simulink model "digital_modlation"  (R2025a)
settings: Solver=VariableStepAuto  StartTime=0.0  StopTime=1  RelTol=1e-3
libraries: dspfdesign x2, commdigbbndpm3 x2, commchan3 x1, commrandsrc3 x1
settings Model: Creator=user  LastModifiedBy=LaL
settings RTWCC: GPUComputeCapability=3.5

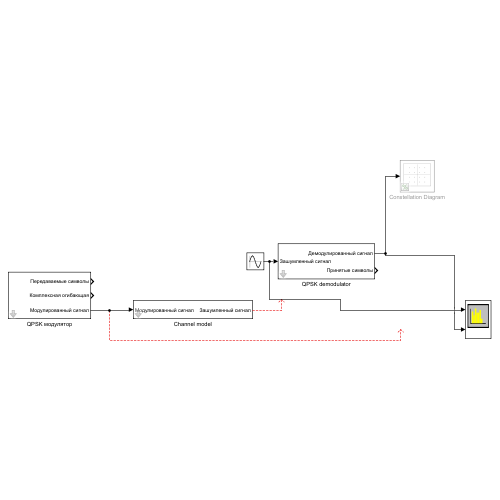
[thumbnail: Simulink's stored preview of the top-level diagram]
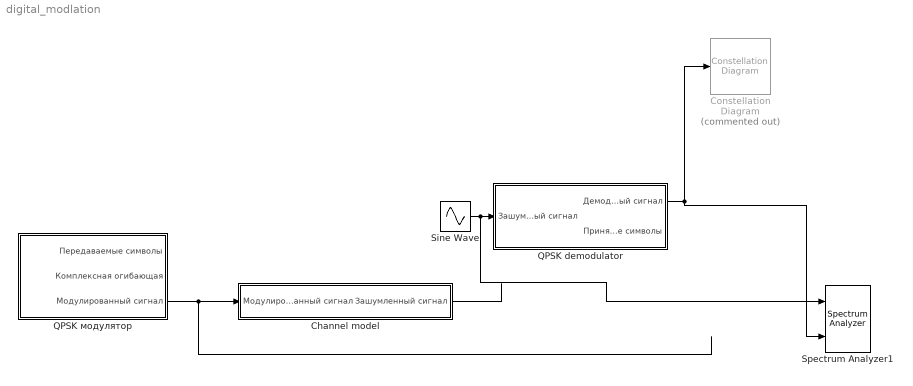
== system digital_modlation ==
  Channel model : Subsystem  mask{SNR=20}
      mask prompts: SNR "SNR (dB)"
  Constellation Diagram : ConstellationDiagram  Commented=on  WindowPosition=[452.000000,103.000000,600.000000,600.000000,]  ScopeFrameLocation=window  SymbolsToDisplaySource=Property  SymbolsToDisplay=300  XLimits=[-1.46,1.46]  YLimits=[-1.38,1.38]  AxesLimits=[-1.38,1.38]  DefaultConfigurationName=comm.scopes.ConstellationDiagramBlockCfg
  QPSK demodulator : Subsystem  mask{symspeed=1000, f=10000, f_d=100000}
      mask prompts: symspeed "Символьная скорость"; f "Частота несущей"; f_d "Частота дискретизации"
  QPSK модулятор : Subsystem  mask{symspeed=1000, f=10000, f_d=100000}
      mask prompts: symspeed "Символьная скорость"; f "Частота несущей"; f_d "Частота дискретизации"
  Sine Wave : Sin  Frequency=10000
  Spectrum Analyzer1 : SpectrumAnalyzer  NumInputPorts=2  WindowPosition=[495.000000,168.000000,800.000000,500.000000,]  Visible=on  ScopeFrameLocation=window  Span=99999.99999999999  StartFrequency=-49999.99999999999  StopFrequency=49999.99999999999  YLimits=[-236.26963761,59.54612507]  SelectedToolstripTab=spectrumAnalyzerToolstrip.measurementsTab
  wires:
  QPSK модулятор/3(Модулированный сигнал) -> Channel model/1(Модулированный сигнал)
  Channel model/1(Зашумленный сигнал) -> ?
  QPSK demodulator/1(Демодулированный сигнал) -> Constellation Diagram/1, Spectrum Analyzer1/2
  Sine Wave/1 -> Spectrum Analyzer1/1, QPSK demodulator/1(Зашумленный сигнал)

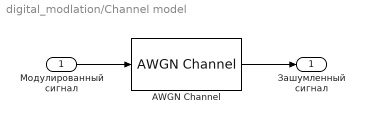
== system digital_modlation/Channel model ==
  Модулированный сигнал : Inport
  AWGN Channel : commchan3/AWGN Channel  LegacyMode=off  NoiseMethod="Signal to noise ratio  (SNR)"  noiseMode="Signal to noise ratio  (SNR)"  EbNo=10  EsNo=10  SNR=SNR  BitsPerSymbol=1  SignalPower=1  SamplesPerSymbol=1  SymbolPeriod=1  VarianceSource=Parameter  Variance=1  RandomStream=Global stream  Seed=67  SimulateUsing=Code generation
  Зашумленный сигнал : Outport
  wires:
  Модулированный сигнал/1 -> AWGN Channel/1
  AWGN Channel/1 -> Зашумленный сигнал/1

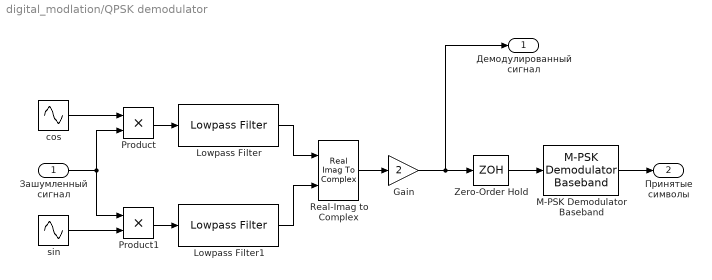
== system digital_modlation/QPSK demodulator ==
  Зашумленный сигнал : Inport
  Gain : Gain  Gain=2
  Lowpass Filter : dspfdesign/Lowpass Filter  FilterType=FIR  DesignForMinimumOrder=on  FilterOrder=50  PassbandFrequency=f  StopbandFrequency=1.2*f  PassbandRipple=0.1  StopbandAttenuation=80  SampleRateMode=Specify on dialog  SampleRate=f_d  SimulateUsing=Interpreted execution  roundingMode=Floor  coeffsDataTypeStr=fixdt(1,16)
  Lowpass Filter1 : dspfdesign/Lowpass Filter  FilterType=FIR  DesignForMinimumOrder=on  FilterOrder=50  PassbandFrequency=f  StopbandFrequency=1.2*f  PassbandRipple=0.1  StopbandAttenuation=80  SampleRateMode=Specify on dialog  SampleRate=f_d  SimulateUsing=Interpreted execution  roundingMode=Floor  coeffsDataTypeStr=fixdt(1,16)
  M-PSK Demodulator Baseband : commdigbbndpm3/M-PSK Demodulator Baseband  M=4  OutType=Integer  DecType=Hard decision  VarSource=Dialog  Variance=1  Dec=Gray  Mapping=[0:7]  Ph=pi/4  outDtype1=Inherit via internal rule  outDtype2=Inherit via internal rule  derotateFactorWordLen=16  derotateFactorDataTypeStr=Inherit: Same word length as input  derotateFactorLastDataTypeStr=Inherit: Same word length as input
      settings: LibrarySourceBlock=|
      | commhdldigbbndpm/M-PSK
      | Demodulator
      | Baseband
  Product : Product
  Product1 : Product
  Real-Imag to Complex : RealImagToComplex
  Zero-Order Hold : ZeroOrderHold  SampleTime=1/symspeed
  cos : Sin  Frequency=2*pi*f  Phase=pi/2  SampleTime=1/f_d
  sin : Sin  Frequency=2*pi*f  SampleTime=1/f_d
  Демодулированный сигнал : Outport
  Принятые символы : Outport  Port=2
  wires:
  Зашумленный сигнал/1 -> Product/2, Product1/1
  cos/1 -> Product/1
  sin/1 -> Product1/2
  Product/1 -> Lowpass Filter/1
  Product1/1 -> Lowpass Filter1/1
  Lowpass Filter/1 -> Real-Imag to Complex/1
  Lowpass Filter1/1 -> Real-Imag to Complex/2
  Real-Imag to Complex/1 -> Gain/1
  Gain/1 -> Zero-Order Hold/1, Демодулированный сигнал/1
  Zero-Order Hold/1 -> M-PSK Demodulator Baseband/1
  M-PSK Demodulator Baseband/1 -> Принятые символы/1

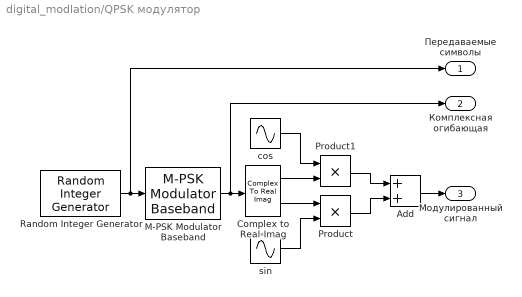
== system digital_modlation/QPSK модулятор ==
  Add : Sum
  Complex to Real-Imag : ComplexToRealImag
  M-PSK Modulator Baseband : commdigbbndpm3/M-PSK Modulator Baseband  M=4  InType=Integer  Enc=Gray  Mapping=[0:7]  Ph=pi/4  outDtype=double  outWordLen=16  outUDDataType=sfix(16)  outFracLenMode=Best precision  outFracLen=15  outDataTypeStr=double  outLastDataTypeStr=double
      settings: LibrarySourceBlock=|
      | commhdldigbbndpm/M-PSK
      | Modulator
      | Baseband
  Product : Product
  Product1 : Product
  Random Integer Generator : commrandsrc3/Random Integer Generator  SetSize=4  SeedSource=Auto  Seed=0  SampleTime=1/symspeed  SamplesPerFrame=1  OutputDataType=uint8  SimulateUsing=Interpreted execution
  cos : Sin  Frequency=2*pi*f  Phase=pi/2  SampleTime=1/f_d
  sin : Sin  Frequency=2*pi*f  SampleTime=1/f_d
  Передаваемые символы : Outport
  Комплексная огибающая : Outport  Port=2
  Модулированный сигнал : Outport  Port=3
  wires:
  Random Integer Generator/1 -> Передаваемые символы/1, M-PSK Modulator Baseband/1
  M-PSK Modulator Baseband/1 -> Комплексная огибающая/1, Complex to Real-Imag/1
  Complex to Real-Imag/1 -> Product1/2
  sin/1 -> Product/2
  cos/1 -> Product1/1
  Complex to Real-Imag/2 -> Product/1
  Product1/1 -> Add/1
  Product/1 -> Add/2
  Add/1 -> Модулированный сигнал/1
